simulink model "odometry_test"  (R2023b)
settings: Solver=VariableStepAuto  StartTime=0.0  StopTime=10.0  MaxStep=0.01  RelTol=1e-3
values from neighbouring files (symbols this model uses):
  Motor_Rev_to_Wheel_Distance = wheel_diameter*pi/gear_ratio    (= 0.0392120947602)    [odometry_data.m]
  Rotation_Local = [1 0 -Distance_FL_y ... (first row only)    [odometry_data.m]
  Rotation_Local_Inv = temp(1:2,:)    [odometry_data.m]
  Wheel_Speed_to_Motor_Speed = 60*gear_ratio/(wheel_diameter*pi)    (= 1530.14013576)    [odometry_data.m]
undefined symbols (not defined in the file or in its folder): DiscIntNeverNeededParam
libraries: simulink_extras x8, simulink x5
settings Model: Creator=ander  LastModifiedBy=ander

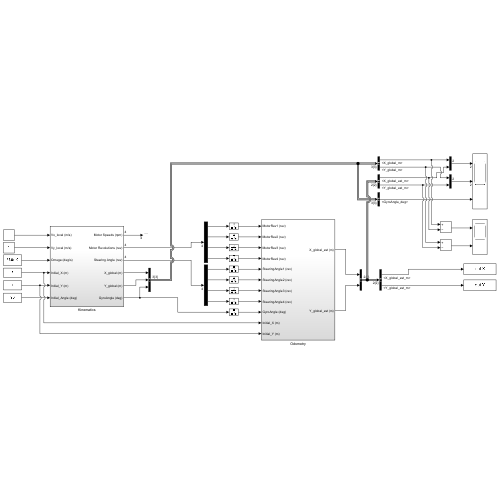
[thumbnail: Simulink's stored preview of the top-level diagram]
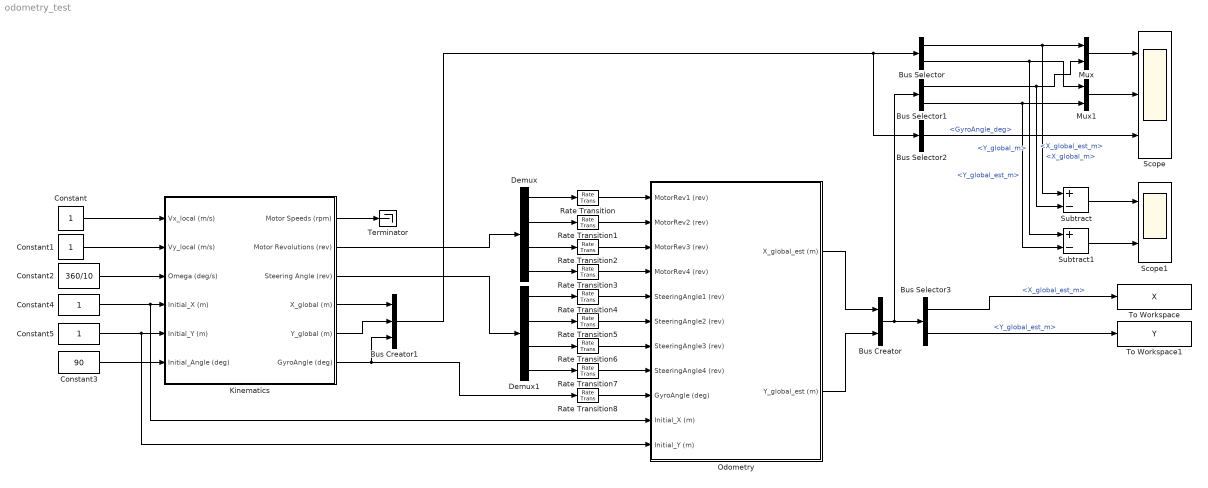
== system odometry_test ==
  Bus Creator : BusCreator  Inputs=2
  Bus Creator1 : BusCreator  Inputs=3
  Bus Selector : BusSelector  OutputSignals=X_global_m,Y_global_m
  Bus Selector1 : BusSelector  OutputSignals=X_global_est_m,Y_global_est_m
  Bus Selector2 : BusSelector  OutputSignals=GyroAngle_deg
  Bus Selector3 : BusSelector  OutputSignals=X_global_est_m,Y_global_est_m
  Constant{,1,4..5} (4 alike) : Constant
  Constant2 : Constant  Value=360/10
  Constant3 : Constant  Value=90
  Demux : Demux
  Demux1 : Demux
  Kinematics : Subsystem
  Mux : Mux  Inputs=2
  Mux1 : Mux  Inputs=2
  Odometry : Subsystem
  Rate Transition{,1..8} (9 alike) : RateTransition  OutPortSampleTime=t_sample
  Scope : Scope  NumInputPorts=3
  Scope1 : Scope  NumInputPorts=2
  Subtract : Sum  Inputs=+-
  Subtract1 : Sum  Inputs=+-
  Terminator : Terminator
  To Workspace : ToWorkspace  VariableName=X  SampleTime=-1
  To Workspace1 : ToWorkspace  VariableName=Y  SampleTime=-1
  wires:
  Kinematics/2(Motor Revolutions (rev)) -> Demux/1
  Kinematics/1(Motor Speeds (rpm)) -> Terminator/1
  Kinematics/3(Steering Angle (rev)) -> Demux1/1
  Demux/3 -> Rate Transition2/1
  Demux/2 -> Rate Transition1/1
  Demux/4 -> Rate Transition3/1
  Demux/1 -> Rate Transition/1
  Demux1/4 -> Rate Transition7/1
  Demux1/3 -> Rate Transition6/1
  Demux1/2 -> Rate Transition5/1
  Demux1/1 -> Rate Transition4/1
  Constant/1 -> Kinematics/1(Vx_local (m/s))
  Constant1/1 -> Kinematics/2(Vy_local (m/s))
  Constant2/1 -> Kinematics/3(Omega (deg/s))
  Constant3/1 -> Kinematics/6(Initial_Angle (deg))
  Kinematics/6(GyroAngle (deg)) -> Bus Creator1/3, Rate Transition8/1
  Rate Transition/1 -> Odometry/1(MotorRev1 (rev))
  Rate Transition1/1 -> Odometry/2(MotorRev2 (rev))
  Rate Transition2/1 -> Odometry/3(MotorRev3 (rev))
  Rate Transition3/1 -> Odometry/4(MotorRev4 (rev))
  Rate Transition4/1 -> Odometry/5(SteeringAngle1 (rev))
  Rate Transition5/1 -> Odometry/6(SteeringAngle2 (rev))
  Rate Transition6/1 -> Odometry/7(SteeringAngle3 (rev))
  Rate Transition7/1 -> Odometry/8(SteeringAngle4 (rev))
  Rate Transition8/1 -> Odometry/9(GyroAngle (deg))
  Mux1/1 -> Scope/2
  Mux/1 -> Scope/1
  Subtract1/1 -> Scope1/2
  Subtract/1 -> Scope1/1
  Constant4/1 -> Odometry/10(Initial_X (m)), Kinematics/4(Initial_X (m))
  Constant5/1 -> Odometry/11(Initial_Y (m)), Kinematics/5(Initial_Y (m))
  Odometry/1(X_global_est (m)) -> Bus Creator/1
  Odometry/2(Y_global_est (m)) -> Bus Creator/2
  Kinematics/4(X_global (m)) -> Bus Creator1/1
  Kinematics/5(Y_global (m)) -> Bus Creator1/2
  Bus Creator1/1 -> Bus Selector2/1, Bus Selector/1
  Bus Selector/1 -> Subtract/1, Mux/1  "<X_global_m>"
  Bus Selector/2 -> Subtract1/1, Mux1/1  "<Y_global_m>"
  Bus Creator/1 -> Bus Selector1/1, Bus Selector3/1
  Bus Selector1/1 -> Subtract/2, Mux/2  "<X_global_est_m>"
  Bus Selector1/2 -> Subtract1/2, Mux1/2  "<Y_global_est_m>"
  Bus Selector2/1 -> Scope/3  "<GyroAngle_deg>"
  Bus Selector3/1 -> To Workspace/1  "<X_global_est_m>"
  Bus Selector3/2 -> To Workspace1/1  "<Y_global_est_m>"

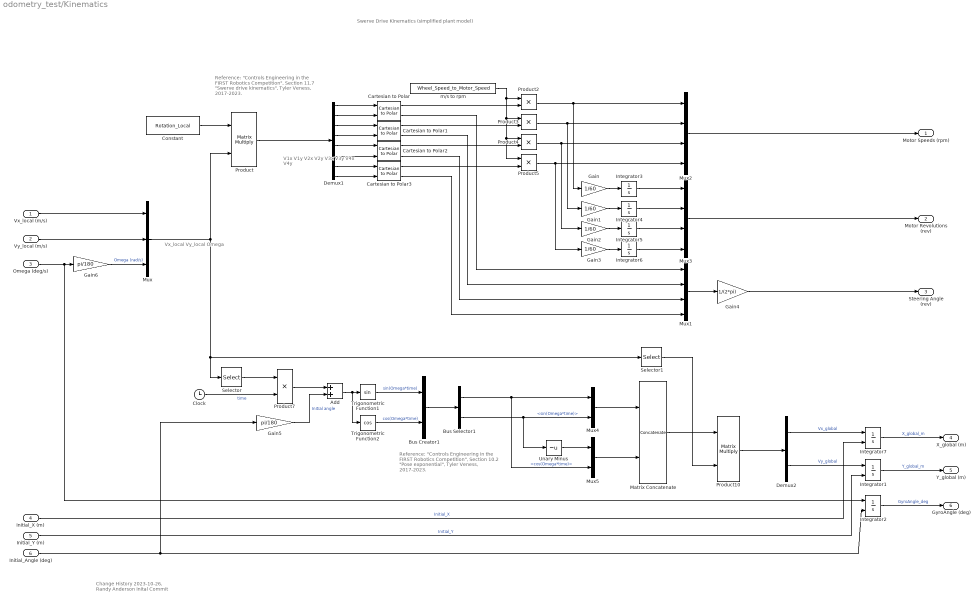
== system odometry_test/Kinematics ==
  note: Swerve Drive Kinematics
      | (simplified plant model)
  note: Vx_local
      | Vy_local
      | Omega
  note: V1x
      | V1y
      | V2x
      | V2y
      | V3x
      | V3y
      | V4x
      | V4y
  note: Reference: "Controls Engineering in the
      |  FIRST Robotics Competition",
      | Section 11.7 "Swerve drive kinematics",
      | Tyler Veness, 2017-2023.
  note: Reference: "Controls Engineering in the
      |  FIRST Robotics Competition",
      | Section 10.2 "Pose exponential",
      | Tyler Veness, 2017-2023.
  note: Change History
      | 2023-10-26, Randy Anderson
      | Inital Commit
  Vx_local (m/s) : Inport
  Vy_local (m/s) : Inport  Port=2
  Omega (deg/s) : Inport  Port=3
  Initial_X (m) : Inport  Port=4
  Initial_Y (m) : Inport  Port=5
  Initial_Angle (deg) : Inport  Port=6
  Add : Sum
  Bus Creator1 : BusCreator  Inputs=2
  Bus Selector1 : BusSelector  OutputSignals=cos(Omega*time),sin(Omega*time)
  Cartesian to Polar{,1..3} (4 alike) : simulink_extras/Transformations/Cartesian to Polar
  Clock : Clock
  Constant : Constant  Value=Rotation_Local
  Demux1 : Demux  Outputs=8
  Demux2 : Demux  Outputs=2
  Gain{,1..3} (4 alike) : Gain  Gain=1/60
  Gain4 : Gain  Gain=1/(2*pi)
  Gain5 : Gain  Gain=pi/180
  Gain6 : Gain  Gain=pi/180
  Integrator1 : Integrator  InitialConditionSource=external
  Integrator2 : Integrator  InitialConditionSource=external
  Integrator{3..6} (4 alike) : Integrator
  Integrator7 : Integrator  InitialConditionSource=external
  Matrix Concatenate : Concatenate  Mode=Multidimensional array  ConcatenateDimension=2
  Mux : Mux  Inputs=3
  Mux1 : Mux
  Mux2 : Mux
  Mux3 : Mux
  Mux4 : Mux  Inputs=2
  Mux5 : Mux  Inputs=2
  Product : Product  Multiplication=Matrix(*)
  Product10 : Product  Multiplication=Matrix(*)
  Product{2..5,7} (5 alike) : Product
  Selector : Selector  InputPortWidth=3  IndexOptions=Index vector (dialog)  Indices=3  OutputSizes=1
  Selector1 : Selector  InputPortWidth=3  IndexOptions=Index vector (dialog)  Indices=[1 2]  OutputSizes=1
  Trigonometric Function1 : Trigonometry
  Trigonometric Function2 : Trigonometry  Operator=cos
  Unary Minus : UnaryMinus
  m/s to rpm : Constant  Value=Wheel_Speed_to_Motor_Speed
  Motor Speeds (rpm) : Outport
  Motor Revolutions (rev) : Outport  Port=2
  Steering Angle (rev) : Outport  Port=3
  X_global (m) : Outport  Port=4
  Y_global (m) : Outport  Port=5
  GyroAngle (deg) : Outport  Port=6
  wires:
  Demux1/2 -> Cartesian to Polar/2
  Integrator6/1 -> Mux3/4
  Integrator5/1 -> Mux3/3
  Product/1 -> Demux1/1
  Cartesian to Polar1/2 -> Mux1/2
  m/s to rpm/1 -> Product5/1, Product4/1, Product3/1, Product2/1
  Constant/1 -> Product/1
  Demux1/8 -> Cartesian to Polar3/2
  Demux1/7 -> Cartesian to Polar3/1
  Demux1/3 -> Cartesian to Polar1/1
  Cartesian to Polar1/1 -> Product3/2
  Mux/1 -> Selector/1, Selector1/1, Product/2
  Mux2/1 -> Motor Speeds (rpm)/1
  Integrator4/1 -> Mux3/2
  Vy_local (m/s)/1 -> Mux/2
  Mux3/1 -> Motor Revolutions (rev)/1
  Gain/1 -> Integrator3/1
  Demux1/1 -> Cartesian to Polar/1
  Cartesian to Polar3/2 -> Mux1/4
  Demux1/5 -> Cartesian to Polar2/1
  Omega (deg/s)/1 -> Integrator2/1, Gain6/1
  Product3/1 -> Gain1/1, Mux2/2
  Cartesian to Polar2/2 -> Mux1/3
  Cartesian to Polar2/1 -> Product4/2
  Product5/1 -> Gain3/1, Mux2/4
  Integrator3/1 -> Mux3/1
  Demux1/4 -> Cartesian to Polar1/2
  Cartesian to Polar/1 -> Product2/2
  Mux1/1 -> Gain4/1
  Vx_local (m/s)/1 -> Mux/1
  Gain2/1 -> Integrator5/1
  Cartesian to Polar/2 -> Mux1/1
  Gain4/1 -> Steering Angle (rev)/1
  Product4/1 -> Gain2/1, Mux2/3
  Product2/1 -> Gain/1, Mux2/1
  Demux1/6 -> Cartesian to Polar2/2
  Cartesian to Polar3/1 -> Product5/2
  Gain1/1 -> Integrator4/1
  Gain3/1 -> Integrator6/1
  Mux4/1 -> Matrix Concatenate/1
  Trigonometric Function1/1 -> Bus Creator1/1  "sin(Omega*time)"
  Trigonometric Function2/1 -> Bus Creator1/2  "cos(Omega*time)"
  Bus Creator1/1 -> Bus Selector1/1
  Mux5/1 -> Matrix Concatenate/2
  Matrix Concatenate/1 -> Product10/1
  Product10/1 -> Demux2/1
  Demux2/1 -> Integrator7/1  "Vx_global"
  Demux2/2 -> Integrator1/1  "Vy_global"
  Bus Selector1/1 -> Mux4/1, Mux5/2  "<cos(Omega*time)>"
  Bus Selector1/2 -> Mux4/2, Unary Minus/1  "<sin(Omega*time)>"
  Unary Minus/1 -> Mux5/1
  Integrator7/1 -> X_global (m)/1  "X_global_m"
  Integrator1/1 -> Y_global (m)/1  "Y_global_m"
  Integrator2/1 -> GyroAngle (deg)/1  "GyroAngle_deg"
  Gain6/1 -> Mux/3  "Omega (rad/s)"
  Clock/1 -> Product7/2  "time"
  Selector/1 -> Product7/1
  Selector1/1 -> Product10/2
  Add/1 -> Trigonometric Function2/1, Trigonometric Function1/1
  Product7/1 -> Add/1
  Gain5/1 -> Add/2  "Initial angle"
  Initial_Angle (deg)/1 -> Gain5/1, Integrator2/2
  Initial_X (m)/1 -> Integrator7/2  "Initial_X"
  Initial_Y (m)/1 -> Integrator1/2  "Initial_Y"

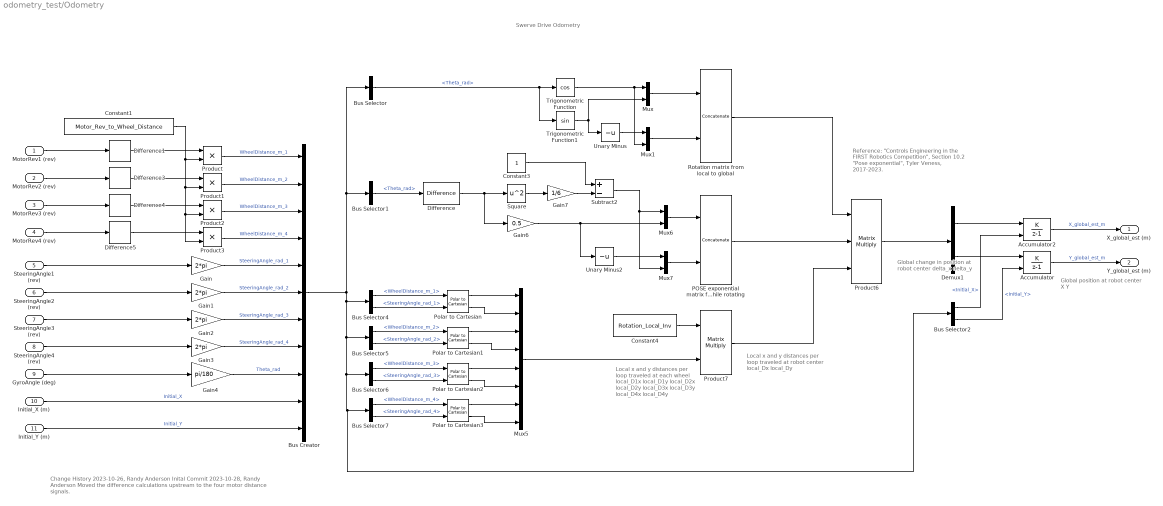
== system odometry_test/Odometry ==
  note: Reference: "Controls Engineering in the
      |  FIRST Robotics Competition",
      | Section 10.2 "Pose exponential",
      | Tyler Veness, 2017-2023.
  note: Local x and y
      | distances per loop
      | traveled at each wheel
      | local_D1x
      | local_D1y
      | local_D2x
      | local_D2y
      | local_D3x
      | local_D3y
      | local_D4x
      | local_D4y
  note: Local x and y
      | distances per loop
      | traveled at robot center
      | local_Dx
      | local_Dy
  note: Global change
      | in position at
      | robot center
      | delta_x
      | delta_y
  note: Global position
      | at robot center
      | X
      | Y
  note: Change History
      | 2023-10-26, Randy Anderson
      | Inital Commit
      | 2023-10-28, Randy Anderson
      | Moved the difference calculations upstream to the four motor distance signals.
  note: Swerve Drive Odometry
  MotorRev1 (rev) : Inport
  MotorRev2 (rev) : Inport  Port=2
  MotorRev3 (rev) : Inport  Port=3
  MotorRev4 (rev) : Inport  Port=4
  SteeringAngle1 (rev) : Inport  Port=5
  SteeringAngle2 (rev) : Inport  Port=6
  SteeringAngle3 (rev) : Inport  Port=7
  SteeringAngle4 (rev) : Inport  Port=8
  GyroAngle (deg) : Inport  Port=9
  Initial_X (m) : Inport  Port=10
  Initial_Y (m) : Inport  Port=11
  Accumulator : DiscreteIntegrator  IntegratorMethod=Accumulation: Forward Euler  InitialConditionSource=external  SampleTime=-1  ICPrevOutput=DiscIntNeverNeededParam  ICPrevScaledInput=DiscIntNeverNeededParam
  Accumulator2 : DiscreteIntegrator  IntegratorMethod=Accumulation: Forward Euler  InitialConditionSource=external  SampleTime=-1  ICPrevOutput=DiscIntNeverNeededParam  ICPrevScaledInput=DiscIntNeverNeededParam
  Bus Creator : BusCreator  Inputs=11
  Bus Selector : BusSelector  OutputSignals=Theta_rad
  Bus Selector1 : BusSelector  OutputSignals=Theta_rad
  Bus Selector2 : BusSelector  OutputSignals=Initial_X,Initial_Y
  Bus Selector4 : BusSelector  OutputSignals=WheelDistance_m_1,SteeringAngle_rad_1
  Bus Selector5 : BusSelector  OutputSignals=WheelDistance_m_2,SteeringAngle_rad_2
  Bus Selector6 : BusSelector  OutputSignals=WheelDistance_m_3,SteeringAngle_rad_3
  Bus Selector7 : BusSelector  OutputSignals=WheelDistance_m_4,SteeringAngle_rad_4
  Constant1 : Constant  Value=Motor_Rev_to_Wheel_Distance
  Constant3 : Constant
  Constant4 : Constant  Value=Rotation_Local_Inv
  Demux1 : Demux  Outputs=2
  Difference{,1,3..5} (5 alike) : simulink/Discrete/Difference  ICPrevInput=0.0  OutMin=[]  OutMax=[]  OutDataType=fixdt(1, 16)  OutScaling=2^-10  DoSatur=off
  Gain{,1..3} (4 alike) : Gain  Gain=2*pi
  Gain4 : Gain  Gain=pi/180
  Gain6 : Gain  Gain=0.5
  Gain7 : Gain  Gain=1/6
  Mux{,1,6..7} (4 alike) : Mux  Inputs=2
  Mux5 : Mux  Inputs=8
  POSE exponential matrix for improved accuracy while rotating : Concatenate  Mode=Multidimensional array  ConcatenateDimension=2
  Polar to Cartesian{,1..3} (4 alike) : simulink_extras/Transformations/Polar to Cartesian
  Product{,1..3} (4 alike) : Product
  Product6 : Product  Inputs=3  Multiplication=Matrix(*)
  Product7 : Product  Multiplication=Matrix(*)
  Rotation matrix from local to global : Concatenate  Mode=Multidimensional array  ConcatenateDimension=2
  Square : Math  Operator=square
  Subtract2 : Sum  Inputs=+-
  Trigonometric Function : Trigonometry  Operator=cos
  Trigonometric Function1 : Trigonometry
  Unary Minus : UnaryMinus
  Unary Minus2 : UnaryMinus
  X_global_est (m) : Outport
  Y_global_est (m) : Outport  Port=2
  wires:
  GyroAngle (deg)/1 -> Gain4/1
  SteeringAngle1 (rev)/1 -> Gain/1
  SteeringAngle2 (rev)/1 -> Gain1/1
  SteeringAngle3 (rev)/1 -> Gain2/1
  SteeringAngle4 (rev)/1 -> Gain3/1
  MotorRev1 (rev)/1 -> Difference1/1
  MotorRev2 (rev)/1 -> Difference3/1
  MotorRev3 (rev)/1 -> Difference4/1
  MotorRev4 (rev)/1 -> Difference5/1
  Product/1 -> Bus Creator/1  "WheelDistance_m_1"
  Product1/1 -> Bus Creator/2  "WheelDistance_m_2"
  Product2/1 -> Bus Creator/3  "WheelDistance_m_3"
  Product3/1 -> Bus Creator/4  "WheelDistance_m_4"
  Constant1/1 -> Product3/2, Product2/2, Product1/2, Product/2
  Gain/1 -> Bus Creator/5  "SteeringAngle_rad_1"
  Gain1/1 -> Bus Creator/6  "SteeringAngle_rad_2"
  Gain2/1 -> Bus Creator/7  "SteeringAngle_rad_3"
  Gain3/1 -> Bus Creator/8  "SteeringAngle_rad_4"
  Bus Creator/1 -> Bus Selector2/1, Bus Selector7/1, Bus Selector6/1, Bus Selector5/1, Bus Selector4/1, Bus Selector/1, Bus Selector1/1
  Bus Selector/1 -> Trigonometric Function1/1, Trigonometric Function/1  "<Theta_rad>"
  Trigonometric Function/1 -> Mux1/2, Mux/1
  Trigonometric Function1/1 -> Unary Minus/1, Mux/2
  Unary Minus/1 -> Mux1/1
  Mux/1 -> Rotation matrix from local to global/1
  Mux1/1 -> Rotation matrix from local to global/2
  Bus Selector1/1 -> Difference/1  "<Theta_rad>"
  Gain4/1 -> Bus Creator/9  "Theta_rad"
  Rotation matrix from local to global/1 -> Product6/1
  Product7/1 -> Product6/3
  Bus Selector4/1 -> Polar to Cartesian/1  "<WheelDistance_m_1>"
  Bus Selector4/2 -> Polar to Cartesian/2  "<SteeringAngle_rad_1>"
  Bus Selector5/2 -> Polar to Cartesian1/2  "<SteeringAngle_rad_2>"
  Bus Selector5/1 -> Polar to Cartesian1/1  "<WheelDistance_m_2>"
  Bus Selector6/1 -> Polar to Cartesian2/1  "<WheelDistance_m_3>"
  Bus Selector6/2 -> Polar to Cartesian2/2  "<SteeringAngle_rad_3>"
  Bus Selector7/2 -> Polar to Cartesian3/2  "<SteeringAngle_rad_4>"
  Bus Selector7/1 -> Polar to Cartesian3/1  "<WheelDistance_m_4>"
  Polar to Cartesian/1 -> Mux5/1
  Polar to Cartesian/2 -> Mux5/2
  Polar to Cartesian1/2 -> Mux5/4
  Polar to Cartesian1/1 -> Mux5/3
  Polar to Cartesian2/2 -> Mux5/6
  Polar to Cartesian2/1 -> Mux5/5
  Polar to Cartesian3/2 -> Mux5/8
  Polar to Cartesian3/1 -> Mux5/7
  Constant4/1 -> Product7/1
  Mux5/1 -> Product7/2
  POSE exponential matrix for improved accuracy while rotating/1 -> Product6/2
  Mux6/1 -> POSE exponential matrix for improved accuracy while rotating/1
  Mux7/1 -> POSE exponential matrix for improved accuracy while rotating/2
  Gain6/1 -> Mux6/2, Unary Minus2/1
  Unary Minus2/1 -> Mux7/1
  Square/1 -> Gain7/1
  Gain7/1 -> Subtract2/2
  Constant3/1 -> Subtract2/1
  Subtract2/1 -> Mux7/2, Mux6/1
  Difference/1 -> Square/1, Gain6/1
  Accumulator2/1 -> X_global_est (m)/1  "X_global_est_m"
  Accumulator/1 -> Y_global_est (m)/1  "Y_global_est_m"
  Product6/1 -> Demux1/1
  Demux1/1 -> Accumulator2/1
  Demux1/2 -> Accumulator/1
  Initial_Y (m)/1 -> Bus Creator/11  "Initial_Y"
  Initial_X (m)/1 -> Bus Creator/10  "Initial_X"
  Bus Selector2/1 -> Accumulator2/2  "<Initial_X>"
  Bus Selector2/2 -> Accumulator/2  "<Initial_Y>"
  Difference1/1 -> Product/1
  Difference3/1 -> Product1/1
  Difference4/1 -> Product2/1
  Difference5/1 -> Product3/1
